simulink model "kundur_pv"  (R2023b)
settings: Solver=ode23tb  StartTime=0.0  StopTime=200  MaxStep=1/60  RelTol=1e-3
InitFcn:
  | SolarInverter_Params();
values from neighbouring files (symbols this model uses):
  Fnom = 60    [SolarInverter_Params.m]
  Pnom = 900e6    (= 900000000)    [SolarInverter_Params.m]
  reec_dbd1 = -0.1    [SolarInverter_Params.m]
  reec_dbd2 = 0.1    [SolarInverter_Params.m]
  reec_dPmax = 0.1    [SolarInverter_Params.m]
  reec_dPmin = -0.1    [SolarInverter_Params.m]
  reec_Imax = 1    [SolarInverter_Params.m]
  reec_Iqhl = 1.0    (= 1)    [SolarInverter_Params.m]
  reec_Iqll = -0.4    [SolarInverter_Params.m]
  reec_Kqi = 0.0    (= 0)    [SolarInverter_Params.m]
  reec_Kqp = 0    [SolarInverter_Params.m]
  reec_Kvi = 0.0    (= 0)    [SolarInverter_Params.m]
  reec_Kvp = 0.1    [SolarInverter_Params.m]
  reec_Pmax = 1.0    (= 1)    [SolarInverter_Params.m]
  reec_Pmin = 0    [SolarInverter_Params.m]
  reec_Qmax = 0.435    [SolarInverter_Params.m]
  reec_Qmin = -0.435    [SolarInverter_Params.m]
  reec_Tiq = 0.02    [SolarInverter_Params.m]
  reec_Tp = 0.02    [SolarInverter_Params.m]
  reec_Tpord = 0.1    [SolarInverter_Params.m]
  reec_Trv = 0.01    [SolarInverter_Params.m]
  reec_Vdip = 0.9    [SolarInverter_Params.m]
  reec_Vmax = 1.10    (= 1.1)    [SolarInverter_Params.m]
  reec_Vmin = 0.9    [SolarInverter_Params.m]
  reec_Vup = 1.15    [SolarInverter_Params.m]
  regc_Brkpt = 0.9    [SolarInverter_Params.m]
  regc_Iolim = -1.2    [SolarInverter_Params.m]
  regc_Iqrmax = 999.9    [SolarInverter_Params.m]
  regc_Iqrmin = -999.9    [SolarInverter_Params.m]
  regc_Ivpnt0 = 0.4    [SolarInverter_Params.m]
  regc_Ivpnt1 = 0.8    [SolarInverter_Params.m]
  regc_Khv = 0.0    (= 0)    [SolarInverter_Params.m]
  regc_Lvpl1 = 1.0    (= 1)    [SolarInverter_Params.m]
  regc_Lvplsw = 0    [SolarInverter_Params.m]
  regc_rrpwr = 10    [SolarInverter_Params.m]
  regc_Tfltr = 0.02    [SolarInverter_Params.m]
  regc_Tg = 0.1    [SolarInverter_Params.m]
  regc_Volim = 1.1    [SolarInverter_Params.m]
  regc_Zerox = 0.5    [SolarInverter_Params.m]
  repc_db1 = 0    [SolarInverter_Params.m]
  repc_Ddn = 20    [SolarInverter_Params.m]
  repc_Dup = 0    [SolarInverter_Params.m]
  repc_emax = 999    [SolarInverter_Params.m]
  repc_emin = -999    [SolarInverter_Params.m]
  repc_fdbd1 = 0.01*0    (= 0)    [SolarInverter_Params.m]
  repc_fdbd2 = -0.01*0    (= 0)    [SolarInverter_Params.m]
  repc_femax = 999    [SolarInverter_Params.m]
  repc_femin = -999    [SolarInverter_Params.m]
  repc_Kc = 0.05    [SolarInverter_Params.m]
  repc_Ki = 1.8    [SolarInverter_Params.m]
  repc_Kig = 0.5    [SolarInverter_Params.m]
  repc_Kp = 0.6    [SolarInverter_Params.m]
  repc_Kpg = 0.1    [SolarInverter_Params.m]
  repc_Pmax = 1    [SolarInverter_Params.m]
  repc_Pmin = 0    [SolarInverter_Params.m]
  repc_Qmax = 0.435    [SolarInverter_Params.m]
  repc_Qmin = -0.435    [SolarInverter_Params.m]
  repc_Rc = 0    [SolarInverter_Params.m]
  repc_Tfltr = 0.02    [SolarInverter_Params.m]
  repc_Tft = 0.5    [SolarInverter_Params.m]
  repc_Tfv = 0.8    [SolarInverter_Params.m]
  repc_Tlag = 0.2    [SolarInverter_Params.m]
  repc_Tp = 0.25    [SolarInverter_Params.m]
  repc_Vfrz = 0.7    [SolarInverter_Params.m]
  repc_Xc = 0    [SolarInverter_Params.m]
  Vnom = 230e3    (= 230000)    [SolarInverter_Params.m]
undefined symbols (not defined in the file or in its folder): D1, Delta, FrqControl, gcbh, j, k_fault, k_pulse, pfaref0, PFControl, PlantControl, PQPriority, Pref_pl, QControl, Qref_pl, QVControl, sps_rtmsupport, Vref_pl
libraries: powerlib_extras x24, simulink x13, spsLoadFlowBusLib x12, spsThreePhaseVIMeasurementLib x11, spsThreePhasePISectionLineLib x8, spsThreePhaseTransformerTwoWindingsLib x5, spsThreePhaseParallelRLCLoadLib x4, spsSynchronousMachinepuStandardLib x4, spsExcitationSystemLib x4, spsSteamTurbineandGovernorLib x4, spsGenericPowerSystemStabilizerLib x4, spsControlledCurrentSourceLib x2
(part 3 of 3)

== system kundur_pv/Renewable Grid-Connection/Break P Loop ==
  u : Inport
  Gain2 : Gain  Gain=1/tau
  Integrator2 : Integrator  InitialCondition=1
  Sum3 : Sum  Inputs=|+-
  to PU1 : Gain  Gain=toPU
  to PU7 : Gain  Gain=1/toPU
  y : Outport  VectorParamsAs1DForOutWhenUnconnected=off
  wires:
  Gain2/1 -> Integrator2/1
  Integrator2/1 -> to PU1/1, Sum3/2
  Sum3/1 -> Gain2/1
  u/1 -> to PU7/1
  to PU7/1 -> Sum3/1
  to PU1/1 -> y/1

== system kundur_pv/Renewable Grid-Connection/Break Q Loop ==
  u : Inport
  Gain2 : Gain  Gain=1/tau
  Integrator2 : Integrator
  Sum3 : Sum  Inputs=|+-
  to PU1 : Gain  Gain=toPU
  to PU7 : Gain  Gain=1/toPU
  y : Outport  VectorParamsAs1DForOutWhenUnconnected=off
  wires:
  to PU1/1 -> y/1
  to PU7/1 -> Sum3/1
  u/1 -> to PU7/1
  Sum3/1 -> Gain2/1
  Integrator2/1 -> Sum3/2, to PU1/1
  Gain2/1 -> Integrator2/1

== system kundur_pv/Renewable Grid-Connection/Break V Loop ==
  u : Inport
  Gain2 : Gain  Gain=1/tau
  Integrator2 : Integrator  InitialCondition=1
  Sum3 : Sum  Inputs=|+-
  to PU1 : Gain  Gain=toPU
  to PU7 : Gain  Gain=1/toPU
  y : Outport  VectorParamsAs1DForOutWhenUnconnected=off
  wires:
  Gain2/1 -> Integrator2/1
  Integrator2/1 -> to PU1/1, Sum3/2
  Sum3/1 -> Gain2/1
  u/1 -> to PU7/1
  to PU7/1 -> Sum3/1
  to PU1/1 -> y/1

== system kundur_pv/Renewable Grid-Connection/Clamping Integrator ==
  LVMax : Inport
  e : Inport  Port=2
  Constant : Constant  Value=-inf
  Constant1 : Constant  Value=0
  Integrator1 : Integrator  InitialCondition=1
  Saturation Dynamic : simulink/Discontinuities/Saturation Dynamic  OutMin=[]  OutMax=[]  OutDataTypeStr=Inherit: Same as second input  OutDataType=fixdt(1, 16)  OutScaling=2^-10  DoSatur=off
  Subsystem : Subsystem
  Switch1 : Switch  Criteria=u2 > Threshold  SaturateOnIntegerOverflow=off  InputSameDT=off
  u : Outport  VectorParamsAs1DForOutWhenUnconnected=off
  wires:
  Saturation Dynamic/1 -> u/1  "u"
  Subsystem/1(Clamp) -> Switch1/2
  Constant/1 -> Saturation Dynamic/3
  Switch1/1 -> Integrator1/1
  LVMax/1 -> Subsystem/3(ymax), Saturation Dynamic/1
  Integrator1/1 -> Subsystem/2(preSat), Saturation Dynamic/2
  e/1 -> Subsystem/1(preIntegrator), Switch1/3
  Constant1/1 -> Switch1/1

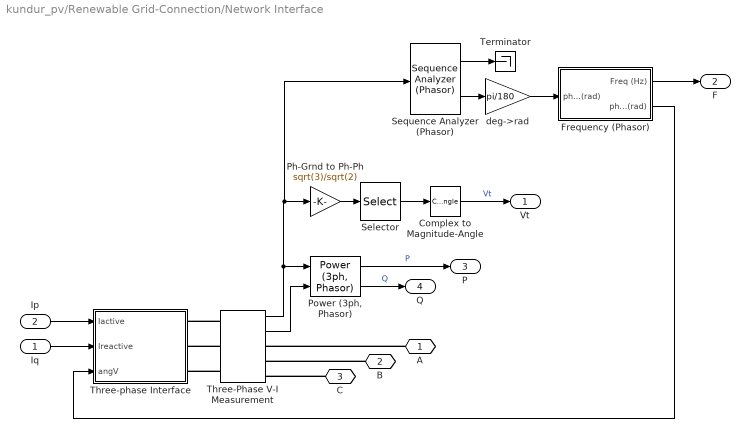
== system kundur_pv/Renewable Grid-Connection/Network Interface ==
  Iq : Inport
  Ip : Inport  Port=2
  Complex to Magnitude-Angle : ComplexToMagnitudeAngle  Output=Magnitude
  Frequency (Phasor) : Subsystem  DialogController=POWERSYS.PowerSysDialog  LoadFcn=sps_rtmsupport('LoadFcn', gcbh);  StartFcn=sps_rtmsupport('StartFcn', gcbh);  StopFcn=sps_rtmsupport('StopFcn', gcbh);  mask(Frequency (Phasor)){Fn=Fnom, T=0.01}
      mask prompts: Fn "Nominal frequency (Hz):"; T "Time constant T for derivative (s):"
      mask help:
      | Frequency is computed by derivative of input phase angle variation with respect to a synchronous phasor rotating at nominal frequency, using the following transfer function:
      |
      |      Hd = s / (1+T.s)
      |
      | The unwraped phase angle (without 2*pi discontinuities) is available at output 2.
      settings: CopyFcn=sps_rtmsupport('CopyFcn', gcbh);  DeleteFcn=sps_rtmsupport('DeleteFcn', gcbh);  UndoDeleteFcn=sps_rtmsupport('UndoDeleteFcn', gcbh);  ModelCloseFcn=sps_rtmsupport('ModelCloseFcn', gcbh);  PreSaveFcn=sps_rtmsupport('PreSaveFcn', gcbh);  PostSaveFcn=sps_rtmsupport('PostSaveFcn', gcbh);  NameChangeFcn=sps_rtmsupport('NameChangeFcn', gcbh);  PreCopyFcn=sps_rtmsupport('PreCopyFcn', gcbh);  OpenFcn=sps_rtmsupport('OpenFcn', gcbh, []);  CloseFcn=sps_rtmsupport('CloseFcn', gcbh);  PreDeleteFcn=sps_rtmsupport('PreDeleteFcn', gcbh);
      mask Help: helpview(psbhelp);
      mask Display:
      | port_label('input',1,'Phase (rad)')
      | port_label('output',1,'Freq (Hz)')
      | port_label('output',2,'\DeltaPhi (rad)', 'texmode', 'on')
  Ph-Grnd to Ph-Ph : Gain  Gain=sqrt(3)/sqrt(2)
  "Power (3ph, Phasor)" : spsPower3phPhasorLib/Power (3ph, Phasor)
      settings: LibrarySourceBlock=|
      | sps_lib/Sensors and Measurements/Power
      | (3ph, Phasor)
  Selector : Selector  InputPortWidth=3  IndexOptions=Index vector (dialog)  Indices=[1]  OutputSizes=1
  Sequence Analyzer (Phasor) : spsSequenceAnalyzerPhasorLib/Sequence Analyzer (Phasor)  seq=Positive
      settings: LibrarySourceBlock=|
      | sps_lib/Sensors and Measurements/Sequence Analyzer
      | (Phasor)
  Terminator : Terminator
  Three-Phase V-I Measurement : spsThreePhaseVIMeasurementLib/Three-Phase V-I Measurement  VoltageMeasurement=phase-to-ground  SetLabelV=off  LabelV=Vabc  Vpu=off  VpuLL=on  CurrentMeasurement=yes  SetLabelI=off  LabelI=Iabc  Ipu=off  Pbase=Pnom  Vbase=Vnom  OutputType=Complex  PhasorSimulation=on  PSBequivalent=0
  Three-phase Interface : Subsystem
  deg->rad : Gain  Gain=pi/180
  A : PMIOPort  Side=Right
  B : PMIOPort  Port=2  Side=Right
  C : PMIOPort  Port=3  Side=Right
  Vt : Outport  VectorParamsAs1DForOutWhenUnconnected=off
  F : Outport  Port=2  VectorParamsAs1DForOutWhenUnconnected=off
  P : Outport  Port=3  VectorParamsAs1DForOutWhenUnconnected=off
  Q : Outport  Port=4  VectorParamsAs1DForOutWhenUnconnected=off
  wires:
  Three-Phase V-I Measurement/1 -> "Power (3ph, Phasor)"/1, Sequence Analyzer (Phasor)/1, Ph-Grnd to Ph-Ph/1
  Three-Phase V-I Measurement/2 -> "Power (3ph, Phasor)"/2
  Selector/1 -> Complex to Magnitude-Angle/1
  Iq/1 -> Three-phase Interface/2(Ireactive)
  Ph-Grnd to Ph-Ph/1 -> Selector/1
  Complex to Magnitude-Angle/1 -> Vt/1  "Vt"
  "Power (3ph, Phasor)"/1 -> P/1  "P"
  Ip/1 -> Three-phase Interface/1(Iactive)
  "Power (3ph, Phasor)"/2 -> Q/1  "Q"
  Sequence Analyzer (Phasor)/2 -> deg->rad/1
  Sequence Analyzer (Phasor)/1 -> Terminator/1
  deg->rad/1 -> Frequency (Phasor)/1(phase (rad))
  Frequency (Phasor)/1(Freq (Hz)) -> F/1
  Frequency (Phasor)/2("phase (rad) ") -> Three-phase Interface/3(angV)
  connections:
  Three-Phase V-I Measurement/LConn3 -- Three-phase Interface/RConn3
  B/RConn1 -- Three-Phase V-I Measurement/RConn2
  Three-Phase V-I Measurement/LConn1 -- Three-phase Interface/RConn1
  A/RConn1 -- Three-Phase V-I Measurement/RConn1
  C/RConn1 -- Three-Phase V-I Measurement/RConn3
  Three-Phase V-I Measurement/LConn2 -- Three-phase Interface/RConn2

== system kundur_pv/Renewable Grid-Connection/Q Current Filter ==
  u : Inport
  1/(taus+1) : Subsystem  mask{tau=tau, vmax=vmax, vmin=vmin}
      mask prompts: tau "Time Constant"
  k : Gain  Gain=k
  y : Outport  VectorParamsAs1DForOutWhenUnconnected=off
  wires:
  1/(taus+1)/1(y) -> y/1
  u/1 -> k/1
  k/1 -> 1/(taus+1)/1(u)

== system kundur_pv/Renewable Grid-Connection/Voltage Filter ==
  u : Inport
  1/(taus+1) : Subsystem  mask{tau=tau, vmax=vmax, vmin=vmin}
      mask prompts: tau "Time Constant"
  k : Gain  Gain=k
  y : Outport  VectorParamsAs1DForOutWhenUnconnected=off
  wires:
  k/1 -> 1/(taus+1)/1(u)
  u/1 -> k/1
  1/(taus+1)/1(y) -> y/1

== system kundur_pv/Utility-scale Solar Electrical Controller/Active Power Filter ==
  u : Inport
  1/(taus+1) : Subsystem  mask{tau=tau, vmax=vmax, vmin=vmin}
      mask prompts: tau "Time Constant"
  k : Gain  Gain=k
  y : Outport  VectorParamsAs1DForOutWhenUnconnected=off
  wires:
  k/1 -> 1/(taus+1)/1(u)
  u/1 -> k/1
  1/(taus+1)/1(y) -> y/1

== system kundur_pv/Utility-scale Solar Electrical Controller/Current Controller ==
  e : Inport
  umax : Inport  Port=2
  umin : Inport  Port=3
  Vdip : Inport  Port=4
  Constant1 : Constant  Value=0
  Display : Display
  Gain : Gain  Gain=Kvp
  Gain1 : Gain  Gain=Kvi
  Integrator1 : Integrator
  OR : Logic  Operator=OR  AllPortsSameDT=off  OutDataTypeStr=boolean
  Saturation Dynamic : simulink/Discontinuities/Saturation Dynamic  OutMin=[]  OutMax=[]  OutDataTypeStr=Inherit: Same as second input  OutDataType=fixdt(1, 16)  OutScaling=2^-10  DoSatur=off
  Subsystem : Subsystem
  Sum1 : Sum  Inputs=++|
  Switch1 : Switch  Criteria=u2 > Threshold  SaturateOnIntegerOverflow=off  InputSameDT=off
  u : Outport  VectorParamsAs1DForOutWhenUnconnected=off
  wires:
  Gain/1 -> Sum1/1
  e/1 -> Gain/1, Gain1/1  "e"
  Constant1/1 -> Switch1/1
  umax/1 -> Subsystem/3(ymax), Saturation Dynamic/1
  Integrator1/1 -> Display/1, Sum1/2
  Gain1/1 -> Subsystem/1(preIntegrator), Switch1/3
  Switch1/1 -> Integrator1/1
  Saturation Dynamic/1 -> u/1  "u"
  Sum1/1 -> Subsystem/2(preSat), Saturation Dynamic/2
  umin/1 -> Subsystem/4(ymin), Saturation Dynamic/3
  Vdip/1 -> OR/1
  Subsystem/1(Clamp) -> OR/2
  OR/1 -> Switch1/2

== system kundur_pv/Utility-scale Solar Electrical Controller/Current Filter ==
  u : Inport
  Vflag : Inport  Port=2
  1/(taus+1) : Subsystem  mask{tau=tau, vmax=vmax, vmin=vmin}
      mask prompts: tau "Time Constant"
  k : Gain  Gain=k
  y : Outport  VectorParamsAs1DForOutWhenUnconnected=off
  wires:
  1/(taus+1)/1(y) -> y/1
  u/1 -> k/1
  k/1 -> 1/(taus+1)/1(u)
  Vflag/1 -> 1/(taus+1)/2(Vflag)

== system kundur_pv/Utility-scale Solar Electrical Controller/P Priority ==
  Ipcmd : Inport
  Constant8 : Constant  Value=Imax
  Sqrt : Sqrt
  Square : Math  Operator=square  SignedPower=on
  Square1 : Math  Operator=square  SignedPower=on
  Sum2 : Sum  Inputs=|+-
  Iqmax : Outport  VectorParamsAs1DForOutWhenUnconnected=off
  wires:
  Sqrt/1 -> Iqmax/1
  Sum2/1 -> Sqrt/1
  Constant8/1 -> Square/1
  Square1/1 -> Sum2/2
  Square/1 -> Sum2/1
  Ipcmd/1 -> Square1/1

== system kundur_pv/Utility-scale Solar Electrical Controller/Q Priority ==
  Iqcmd : Inport
  Constant8 : Constant  Value=Imax
  Sqrt : Sqrt
  Square : Math  Operator=square  SignedPower=on
  Square1 : Math  Operator=square  SignedPower=on
  Sum2 : Sum  Inputs=|+-
  Ipmax : Outport  VectorParamsAs1DForOutWhenUnconnected=off
  wires:
  Sqrt/1 -> Ipmax/1
  Sum2/1 -> Sqrt/1
  Constant8/1 -> Square/1
  Square1/1 -> Sum2/2
  Square/1 -> Sum2/1
  Iqcmd/1 -> Square1/1

== system kundur_pv/Utility-scale Solar Electrical Controller/Reference Power Filter ==
  u : Inport
  Vflag : Inport  Port=2
  1/(taus+1) : Subsystem  mask{tau=tau, vmax=vmax, vmin=vmin}
      mask prompts: tau "Time Constant"
  k : Gain  Gain=k
  y : Outport  VectorParamsAs1DForOutWhenUnconnected=off
  wires:
  Vflag/1 -> 1/(taus+1)/2(Vflag)
  k/1 -> 1/(taus+1)/1(u)
  u/1 -> k/1
  1/(taus+1)/1(y) -> y/1

== system kundur_pv/Utility-scale Solar Electrical Controller/Vref0 ==
  Constant6 : Constant  Value=0
  Init_Val : Integrator  InitialCondition=1
  Vref0 : Outport  VectorParamsAs1DForOutWhenUnconnected=off
  wires:
  Constant6/1 -> Init_Val/1
  Init_Val/1 -> Vref0/1

== system kundur_pv/Utility-scale Solar Electrical Controller/Vt Filter ==
  u : Inport
  1/(taus+1) : Subsystem  mask{tau=tau, vmax=vmax, vmin=vmin}
      mask prompts: tau "Time Constant"
  k : Gain  Gain=k
  y : Outport  VectorParamsAs1DForOutWhenUnconnected=off
  wires:
  k/1 -> 1/(taus+1)/1(u)
  u/1 -> k/1
  1/(taus+1)/1(y) -> y/1

== system kundur_pv/Utility-scale Solar Electrical Controller/pfaref ==
  Constant1 : Constant  Value=cos(pfaref0)
  Constant6 : Constant  Value=0
  Init_Val : Integrator
  Trigonometric Function : Trigonometry  Operator=acos
  pfaref : Outport  VectorParamsAs1DForOutWhenUnconnected=off
  wires:
  Constant6/1 -> Init_Val/1
  Constant1/1 -> Trigonometric Function/1
  Trigonometric Function/1 -> pfaref/1

== system kundur_pv/Utility-scale Solar Plant Controller/Lag Filter ==
  u : Inport
  1/(taus+1) : Subsystem  mask{tau=tau, vmax=vmax, vmin=vmin}
      mask prompts: tau "Time Constant"
  k : Gain  Gain=k
  y : Outport  VectorParamsAs1DForOutWhenUnconnected=off
  wires:
  k/1 -> 1/(taus+1)/1(u)
  u/1 -> k/1
  1/(taus+1)/1(y) -> y/1

== system kundur_pv/Utility-scale Solar Plant Controller/Lead-Lag ==
  note: disable integrator and pass through signal if tb is zero
  u : Inport
  Constant : Constant  Value=tb
  Gain : Gain  Gain=1/(tb+eps)
  Gain1 : Gain  Gain=ta
  Integrator : Integrator
  Sum : Sum  Inputs=|+-
  Sum1 : Sum  Inputs=++|
  Switch : Switch  Criteria=u2 > Threshold  SaturateOnIntegerOverflow=off  InputSameDT=off
  Switch1 : Switch  Criteria=u2 > Threshold  SaturateOnIntegerOverflow=off  InputSameDT=off
  y : Outport  VectorParamsAs1DForOutWhenUnconnected=off
  wires:
  Sum/1 -> Gain/1
  Gain/1 -> Switch/1, Gain1/1
  Gain1/1 -> Sum1/1
  Integrator/1 -> Sum1/2, Sum/2
  u/1 -> Switch1/3, Sum/1
  Constant/1 -> Switch1/2, Switch/3, Switch/2
  Switch/1 -> Integrator/1
  Sum1/1 -> Switch1/1
  Switch1/1 -> y/1

== system kundur_pv/Utility-scale Solar Plant Controller/P Filter ==
  u : Inport
  1/(taus+1) : Subsystem  mask{tau=tau, vmax=vmax, vmin=vmin}
      mask prompts: tau "Time Constant"
  k : Gain  Gain=k
  y : Outport  VectorParamsAs1DForOutWhenUnconnected=off
  wires:
  k/1 -> 1/(taus+1)/1(u)
  u/1 -> k/1
  1/(taus+1)/1(y) -> y/1

== system kundur_pv/Utility-scale Solar Plant Controller/Q Filter ==
  u : Inport
  1/(taus+1) : Subsystem  mask{tau=tau, vmax=vmax, vmin=vmin}
      mask prompts: tau "Time Constant"
  k : Gain  Gain=k
  y : Outport  VectorParamsAs1DForOutWhenUnconnected=off
  wires:
  k/1 -> 1/(taus+1)/1(u)
  u/1 -> k/1
  1/(taus+1)/1(y) -> y/1

== system kundur_pv/Utility-scale Solar Plant Controller/Reactive Power Controller ==
  e : Inport
  Frz : Inport  Port=2
  Constant : Constant  Value=Qmax
  Constant1 : Constant  Value=0
  Constant2 : Constant  Value=Qmin
  Display2 : Display
  Gain : Gain  Gain=Kp
  Gain1 : Gain  Gain=Ki
  Integrator1 : Integrator
  OR : Logic  Operator=OR  AllPortsSameDT=off  OutDataTypeStr=boolean
  Saturation Dynamic : simulink/Discontinuities/Saturation Dynamic  OutMin=[]  OutMax=[]  OutDataTypeStr=Inherit: Same as second input  OutDataType=fixdt(1, 16)  OutScaling=2^-10  DoSatur=off
  Subsystem : Subsystem
  Sum1 : Sum  Inputs=++|
  Switch1 : Switch  Criteria=u2 > Threshold  SaturateOnIntegerOverflow=off  InputSameDT=off
  u : Outport  VectorParamsAs1DForOutWhenUnconnected=off
  wires:
  OR/1 -> Switch1/2
  Subsystem/1(Clamp) -> OR/2
  Frz/1 -> OR/1
  Constant2/1 -> Saturation Dynamic/3, Subsystem/4(ymin)
  Sum1/1 -> Display2/1, Saturation Dynamic/2, Subsystem/2(preSat)
  Saturation Dynamic/1 -> u/1  "u"
  Switch1/1 -> Integrator1/1
  Gain1/1 -> Switch1/3, Subsystem/1(preIntegrator)
  Integrator1/1 -> Sum1/2
  Constant/1 -> Saturation Dynamic/1, Subsystem/3(ymax)
  Constant1/1 -> Switch1/1
  e/1 -> Gain1/1, Gain/1  "e"
  Gain/1 -> Sum1/1

== system kundur_pv/Utility-scale Solar Plant Controller/Subsystem ==
  Ibranch : Inport
  Vreg : Inport  Port=2
  Complex to Magnitude : ComplexToMagnitudeAngle  Output=Magnitude
  Gain : Gain  Gain=Rc
  Gain1 : Gain  Gain=j*Xc
  Sum : Sum  Inputs=|++
  Sum1 : Sum  Inputs=|-+
  Ve : Outport  VectorParamsAs1DForOutWhenUnconnected=off
  wires:
  Ibranch/1 -> Gain/1, Gain1/1
  Gain/1 -> Sum/1
  Vreg/1 -> Sum1/2
  Sum/1 -> Sum1/1
  Gain1/1 -> Sum/2
  Sum1/1 -> Complex to Magnitude/1
  Complex to Magnitude/1 -> Ve/1  "Ve"

== system kundur_pv/Utility-scale Solar Plant Controller/Vcomp Filter ==
  u : Inport
  1/(taus+1) : Subsystem  mask{tau=tau, vmax=vmax, vmin=vmin}
      mask prompts: tau "Time Constant"
  k : Gain  Gain=k
  y : Outport  VectorParamsAs1DForOutWhenUnconnected=off
  wires:
  k/1 -> 1/(taus+1)/1(u)
  u/1 -> k/1
  1/(taus+1)/1(y) -> y/1

== system kundur_pv/Renewable Grid-Connection/Clamping Integrator/Subsystem ==
  preIntegrator : Inport
  preSat : Inport  Port=2
  ymax : Inport  Port=3
  AND1 : Logic  AllPortsSameDT=off  OutDataTypeStr=boolean
  Constant : Constant  Value=-inf
  Data Type Conversion : DataTypeConversion  OutDataTypeStr=int8  SaturateOnIntegerOverflow=off  RndMeth=Floor
  Data Type Conversion1 : DataTypeConversion  OutDataTypeStr=int8  SaturateOnIntegerOverflow=off  RndMeth=Floor
  Dead Zone Dynamic : simulink/Discontinuities/Dead Zone Dynamic
  Equal1 : RelationalOperator  Operator===  OutDataTypeStr=boolean  RndMeth=Simplest  InputSameDT=off
  Gain2 : Gain  Gain=0
  Memory1 : Memory
  Relational Operator : RelationalOperator  Operator=~=  OutDataTypeStr=boolean  RndMeth=Simplest  InputSameDT=off
  Sign : Signum
  Sign1 : Signum
  Clamp : Outport  VectorParamsAs1DForOutWhenUnconnected=off
  wires:
  Sign/1 -> Data Type Conversion/1
  AND1/1 -> Memory1/1
  Dead Zone Dynamic/1 -> Relational Operator/2, Sign/1
  Data Type Conversion/1 -> Equal1/1
  Gain2/1 -> Relational Operator/1
  Equal1/1 -> AND1/2
  preSat/1 -> Dead Zone Dynamic/2, Gain2/1
  Relational Operator/1 -> AND1/1
  Sign1/1 -> Data Type Conversion1/1
  preIntegrator/1 -> Sign1/1
  Data Type Conversion1/1 -> Equal1/2
  ymax/1 -> Dead Zone Dynamic/1
  Constant/1 -> Dead Zone Dynamic/3
  Memory1/1 -> Clamp/1  "Clamp"

== system kundur_pv/Renewable Grid-Connection/Network Interface/Frequency (Phasor) ==
  phase (rad) : Inport
  " Wn" : Constant  Value=Fn*2*pi
  Add : Sum
  IC : InitialCondition  Commented=through  Value=0
  Unit Delay : UnitDelay  SampleTime=-1  HasFrameUpgradeWarning=on
  Unit Delay1 : UnitDelay  SampleTime=-1  HasFrameUpgradeWarning=on
  derivative : TransferFcn  Numerator="[1  0]"  Denominator="[T  1]"
  if structure : MATLAB Function  TreatAsAtomicUnit=on
  rad/s to Hz : Gain  Gain=1/(2*pi)
  Freq (Hz) : Outport  VectorParamsAs1DForOutWhenUnconnected=off
  "phase (rad) " : Outport  Port=2  VectorParamsAs1DForOutWhenUnconnected=off
  wires:
  Add/1 -> rad/s to Hz/1
  if structure/1(y) -> Unit Delay/1, derivative/1, "phase (rad) "/1
  rad/s to Hz/1 -> Freq (Hz)/1
  derivative/1 -> Add/1
  " Wn"/1 -> Add/2
  IC/1 -> if structure/1(phase)
  Unit Delay/1 -> if structure/3(y_old)
  Unit Delay1/1 -> if structure/2(phase_old)
  phase (rad)/1 -> Unit Delay1/1, IC/1

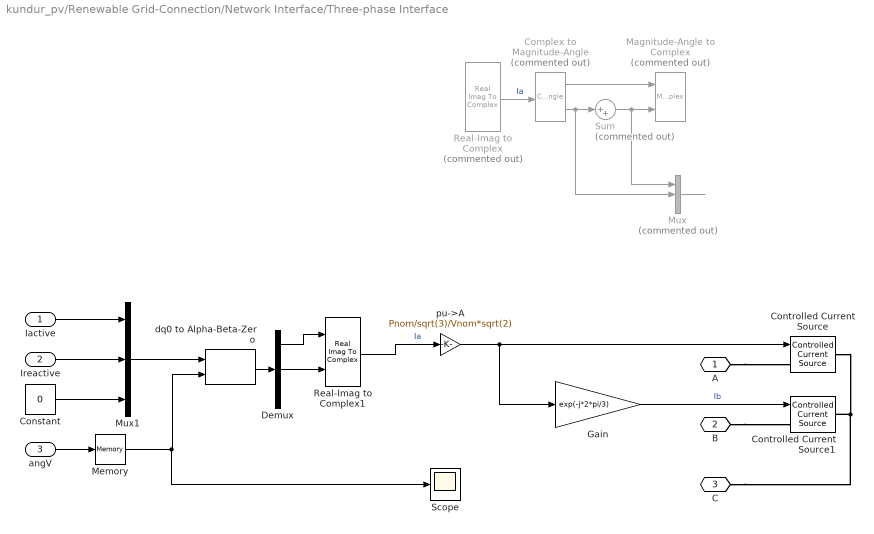
== system kundur_pv/Renewable Grid-Connection/Network Interface/Three-phase Interface ==
  Iactive : Inport
  Ireactive : Inport  Port=2
  angV : Inport  Port=3
  Complex to Magnitude-Angle : ComplexToMagnitudeAngle  Commented=on
  Constant : Constant  Value=0
  Controlled Current Source : spsControlledCurrentSourceLib/Controlled Current Source  Initialize=on  Source_Type=AC  Amplitude=-1*Pnom/sqrt(3)/Vnom*sqrt(2)  Phase=0  Frequency=Fnom  Measurements=None
  Controlled Current Source1 : spsControlledCurrentSourceLib/Controlled Current Source  Initialize=on  Source_Type=AC  Amplitude=-1*Pnom/sqrt(3)/Vnom*sqrt(2)  Phase=120  Frequency=Fnom  Measurements=None
  Demux : Demux  Outputs=3
  Gain : Gain  Gain=exp(-j*2*pi/3)
  Magnitude-Angle to Complex : MagnitudeAngleToComplex  Commented=on
  Memory : Memory  InitialCondition=0.1
  Mux : Mux  Commented=on  Inputs=3
  Mux1 : Mux  Inputs=3
  Real-Imag to Complex : RealImagToComplex  Commented=on
  Real-Imag to Complex1 : RealImagToComplex
  Scope : Scope
  Sum : Sum  Commented=on  Inputs=|++
  dq0 to Alpha-Beta-Zero : spsdq0toAlphaBetaZeroLib/dq0 to Alpha-Beta-Zero  Alignment=Aligned with phase A axis
  "pu->A " : Gain  Gain=Pnom/sqrt(3)/Vnom*sqrt(2)  SaturateOnIntegerOverflow=on  OutDataTypeStr=Inherit: Same as input  ParamDataTypeStr=Inherit: Same as input
  A : PMIOPort  Side=Right
  B : PMIOPort  Port=2  Side=Right
  C : PMIOPort  Port=3  Side=Right
  wires:
  Gain/1 -> Controlled Current Source1/1  "Ib"
  Real-Imag to Complex/1 -> Complex to Magnitude-Angle/1  "Ia"
  Complex to Magnitude-Angle/1 -> Magnitude-Angle to Complex/1
  Complex to Magnitude-Angle/2 -> Mux/2, Sum/1
  Sum/1 -> Mux/1, Magnitude-Angle to Complex/2
  "pu->A "/1 -> Gain/1, Controlled Current Source/1
  Mux/1 -> ?
  angV/1 -> Memory/1
  Iactive/1 -> Mux1/1
  Ireactive/1 -> Mux1/2
  Constant/1 -> Mux1/3
  Mux1/1 -> dq0 to Alpha-Beta-Zero/1
  dq0 to Alpha-Beta-Zero/1 -> Demux/1
  Demux/2 -> Real-Imag to Complex1/2
  Demux/1 -> Real-Imag to Complex1/1
  Real-Imag to Complex1/1 -> "pu->A "/1  "Ia"
  Memory/1 -> Scope/1, dq0 to Alpha-Beta-Zero/2
  connections:
  Controlled Current Source/RConn1 -- C/RConn1 -- Controlled Current Source1/RConn1
  A/RConn1 -- Controlled Current Source/LConn1
  B/RConn1 -- Controlled Current Source1/LConn1

== system kundur_pv/Renewable Grid-Connection/Q Current Filter/1//(taus+1) ==
  note: disable integrator and pass through signal if tau is zero
  u : Inport
  Constant : Constant  Value=tau
  Gain1 : Gain  Gain=1/(tau+eps)  SaturateOnIntegerOverflow=on  OutDataTypeStr=Inherit: Same as input  ParamDataTypeStr=Inherit: Same as input
  Integrator : Integrator  LimitOutput=on  UpperSaturationLimit=vmax  LowerSaturationLimit=vmin
  Sum : Sum  Inputs=|+-  InputSameDT=on  SaturateOnIntegerOverflow=on  OutDataTypeStr=Inherit: Same as first input
  Switch : Switch  Criteria=u2 > Threshold  SaturateOnIntegerOverflow=off  InputSameDT=off
  Switch1 : Switch  Criteria=u2 > Threshold  SaturateOnIntegerOverflow=off  InputSameDT=off
  y : Outport  VectorParamsAs1DForOutWhenUnconnected=off
  wires:
  Switch1/1 -> y/1
  Switch/1 -> Integrator/1
  Gain1/1 -> Switch/1
  Constant/1 -> Switch/2, Switch1/2, Switch/3
  Integrator/1 -> Switch1/1, Sum/2
  Sum/1 -> Gain1/1
  u/1 -> Sum/1, Switch1/3

== system kundur_pv/Renewable Grid-Connection/Voltage Filter/1//(taus+1) ==
  note: disable integrator and pass through signal if tau is zero
  u : Inport
  Constant : Constant  Value=tau
  Gain1 : Gain  Gain=1/(tau+eps)  SaturateOnIntegerOverflow=on  OutDataTypeStr=Inherit: Same as input  ParamDataTypeStr=Inherit: Same as input
  Integrator : Integrator  InitialCondition=1  LimitOutput=on  UpperSaturationLimit=vmax  LowerSaturationLimit=vmin
  Sum : Sum  Inputs=|+-  InputSameDT=on  SaturateOnIntegerOverflow=on  OutDataTypeStr=Inherit: Same as first input
  Switch : Switch  Criteria=u2 > Threshold  SaturateOnIntegerOverflow=off  InputSameDT=off
  Switch1 : Switch  Criteria=u2 > Threshold  SaturateOnIntegerOverflow=off  InputSameDT=off
  y : Outport  VectorParamsAs1DForOutWhenUnconnected=off
  wires:
  Sum/1 -> Gain1/1
  Integrator/1 -> Sum/2, Switch1/1
  Constant/1 -> Switch/3, Switch1/2, Switch/2
  Gain1/1 -> Switch/1
  Switch/1 -> Integrator/1
  Switch1/1 -> y/1
  u/1 -> Switch1/3, Sum/1

== system kundur_pv/Utility-scale Solar Electrical Controller/Active Power Filter/1//(taus+1) ==
  note: disable integrator and pass through signal if tau is zero
  u : Inport
  Constant : Constant  Value=tau
  Gain1 : Gain  Gain=1/(tau+eps)  SaturateOnIntegerOverflow=on  OutDataTypeStr=Inherit: Same as input  ParamDataTypeStr=Inherit: Same as input
  Integrator : Integrator  InitialCondition=1  LimitOutput=on  UpperSaturationLimit=vmax  LowerSaturationLimit=vmin
  Sum : Sum  Inputs=|+-  InputSameDT=on  SaturateOnIntegerOverflow=on  OutDataTypeStr=Inherit: Same as first input
  Switch : Switch  Criteria=u2 > Threshold  SaturateOnIntegerOverflow=off  InputSameDT=off
  Switch1 : Switch  Criteria=u2 > Threshold  SaturateOnIntegerOverflow=off  InputSameDT=off
  y : Outport  VectorParamsAs1DForOutWhenUnconnected=off
  wires:
  u/1 -> Switch1/3, Sum/1
  Sum/1 -> Gain1/1
  Integrator/1 -> Sum/2, Switch1/1
  Constant/1 -> Switch/3, Switch1/2, Switch/2
  Gain1/1 -> Switch/1
  Switch/1 -> Integrator/1
  Switch1/1 -> y/1

== system kundur_pv/Utility-scale Solar Electrical Controller/Current Controller/Subsystem ==
  preIntegrator : Inport
  preSat : Inport  Port=2
  ymax : Inport  Port=3
  ymin : Inport  Port=4
  AND1 : Logic  AllPortsSameDT=off  OutDataTypeStr=boolean
  Data Type Conversion : DataTypeConversion  OutDataTypeStr=int8  SaturateOnIntegerOverflow=off  RndMeth=Floor
  Data Type Conversion1 : DataTypeConversion  OutDataTypeStr=int8  SaturateOnIntegerOverflow=off  RndMeth=Floor
  Dead Zone Dynamic : simulink/Discontinuities/Dead Zone Dynamic
  Equal1 : RelationalOperator  Operator===  OutDataTypeStr=boolean  RndMeth=Simplest  InputSameDT=off
  Gain2 : Gain  Gain=0
  Memory1 : Memory
  Relational Operator : RelationalOperator  Operator=~=  OutDataTypeStr=boolean  RndMeth=Simplest  InputSameDT=off
  Sign : Signum
  Sign1 : Signum
  Clamp : Outport  VectorParamsAs1DForOutWhenUnconnected=off
  wires:
  Sign/1 -> Data Type Conversion/1
  AND1/1 -> Memory1/1
  Dead Zone Dynamic/1 -> Relational Operator/2, Sign/1
  Data Type Conversion/1 -> Equal1/1
  Gain2/1 -> Relational Operator/1
  Equal1/1 -> AND1/2
  preSat/1 -> Dead Zone Dynamic/2, Gain2/1
  Relational Operator/1 -> AND1/1
  Sign1/1 -> Data Type Conversion1/1
  preIntegrator/1 -> Sign1/1
  Data Type Conversion1/1 -> Equal1/2
  ymax/1 -> Dead Zone Dynamic/1
  ymin/1 -> Dead Zone Dynamic/3
  Memory1/1 -> Clamp/1  "Clamp"

== system kundur_pv/Utility-scale Solar Electrical Controller/Current Filter/1//(taus+1) ==
  note: disable integrator and pass through signal if tau is zero
  u : Inport
  Vflag : Inport  Port=2
  Constant : Constant  Value=tau
  Constant1 : Constant  Value=0
  Gain1 : Gain  Gain=1/(tau+eps)  SaturateOnIntegerOverflow=on  OutDataTypeStr=Inherit: Same as input  ParamDataTypeStr=Inherit: Same as input
  Integrator : Integrator  LimitOutput=on  UpperSaturationLimit=vmax  LowerSaturationLimit=vmin
  Subsystem : Subsystem
  Sum : Sum  Inputs=|+-  InputSameDT=on  SaturateOnIntegerOverflow=on  OutDataTypeStr=Inherit: Same as first input
  Switch : Switch  Criteria=u2 > Threshold  SaturateOnIntegerOverflow=off  InputSameDT=off
  Switch1 : Switch  Criteria=u2 > Threshold  SaturateOnIntegerOverflow=off  InputSameDT=off
  y : Outport  VectorParamsAs1DForOutWhenUnconnected=off
  wires:
  Switch1/1 -> y/1
  Switch/1 -> Integrator/1
  Gain1/1 -> Switch/1
  Constant/1 -> Switch1/2, Subsystem/1(tau)
  Integrator/1 -> Switch1/1, Sum/2
  Sum/1 -> Gain1/1
  u/1 -> Sum/1, Switch1/3
  Constant1/1 -> Switch/3
  Subsystem/1(Out1) -> Switch/2
  Vflag/1 -> Subsystem/2(Vflag)

== system kundur_pv/Utility-scale Solar Electrical Controller/Reference Power Filter/1//(taus+1) ==
  note: disable integrator and pass through signal if tau is zero
  u : Inport
  Vflag : Inport  Port=2
  Constant : Constant  Value=tau
  Constant1 : Constant  Value=0
  Gain1 : Gain  Gain=1/(tau+eps)  SaturateOnIntegerOverflow=on  OutDataTypeStr=Inherit: Same as input  ParamDataTypeStr=Inherit: Same as input
  Integrator : Integrator  InitialCondition=0.999  LimitOutput=on  UpperSaturationLimit=vmax  LowerSaturationLimit=vmin
  Subsystem : Subsystem
  Sum : Sum  Inputs=|+-  InputSameDT=on  SaturateOnIntegerOverflow=on  OutDataTypeStr=Inherit: Same as first input
  Switch : Switch  Criteria=u2 > Threshold  SaturateOnIntegerOverflow=off  InputSameDT=off
  Switch1 : Switch  Criteria=u2 > Threshold  SaturateOnIntegerOverflow=off  InputSameDT=off
  y : Outport  VectorParamsAs1DForOutWhenUnconnected=off
  wires:
  Vflag/1 -> Subsystem/2(Vflag)
  Subsystem/1(Out1) -> Switch/2
  Constant1/1 -> Switch/3
  u/1 -> Switch1/3, Sum/1
  Sum/1 -> Gain1/1
  Integrator/1 -> Sum/2, Switch1/1
  Constant/1 -> Subsystem/1(tau), Switch1/2
  Gain1/1 -> Switch/1
  Switch/1 -> Integrator/1
  Switch1/1 -> y/1

== system kundur_pv/Utility-scale Solar Electrical Controller/Vt Filter/1//(taus+1) ==
  note: disable integrator and pass through signal if tau is zero
  u : Inport
  Constant : Constant  Value=tau
  Gain1 : Gain  Gain=1/(tau+eps)  SaturateOnIntegerOverflow=on  OutDataTypeStr=Inherit: Same as input  ParamDataTypeStr=Inherit: Same as input
  Integrator : Integrator  InitialCondition=1  LimitOutput=on  UpperSaturationLimit=vmax  LowerSaturationLimit=vmin
  Sum : Sum  Inputs=|+-  InputSameDT=on  SaturateOnIntegerOverflow=on  OutDataTypeStr=Inherit: Same as first input
  Switch : Switch  Criteria=u2 > Threshold  SaturateOnIntegerOverflow=off  InputSameDT=off
  Switch1 : Switch  Criteria=u2 > Threshold  SaturateOnIntegerOverflow=off  InputSameDT=off
  y : Outport  VectorParamsAs1DForOutWhenUnconnected=off
  wires:
  u/1 -> Switch1/3, Sum/1
  Sum/1 -> Gain1/1
  Integrator/1 -> Sum/2, Switch1/1
  Constant/1 -> Switch/3, Switch1/2, Switch/2
  Gain1/1 -> Switch/1
  Switch/1 -> Integrator/1
  Switch1/1 -> y/1

== system kundur_pv/Utility-scale Solar Plant Controller/Lag Filter/1//(taus+1) ==
  note: disable integrator and pass through signal if tau is zero
  u : Inport
  Constant : Constant  Value=tau
  Gain1 : Gain  Gain=1/(tau+eps)  SaturateOnIntegerOverflow=on  OutDataTypeStr=Inherit: Same as input  ParamDataTypeStr=Inherit: Same as input
  Integrator : Integrator  InitialCondition=1  LimitOutput=on  UpperSaturationLimit=vmax  LowerSaturationLimit=vmin
  Sum : Sum  Inputs=|+-  InputSameDT=on  SaturateOnIntegerOverflow=on  OutDataTypeStr=Inherit: Same as first input
  Switch : Switch  Criteria=u2 > Threshold  SaturateOnIntegerOverflow=off  InputSameDT=off
  Switch1 : Switch  Criteria=u2 > Threshold  SaturateOnIntegerOverflow=off  InputSameDT=off
  y : Outport  VectorParamsAs1DForOutWhenUnconnected=off
  wires:
  u/1 -> Switch1/3, Sum/1
  Sum/1 -> Gain1/1
  Integrator/1 -> Sum/2, Switch1/1
  Constant/1 -> Switch/3, Switch1/2, Switch/2
  Gain1/1 -> Switch/1
  Switch/1 -> Integrator/1
  Switch1/1 -> y/1

== system kundur_pv/Utility-scale Solar Plant Controller/P Filter/1//(taus+1) ==
  note: disable integrator and pass through signal if tau is zero
  u : Inport
  Constant : Constant  Value=tau
  Gain1 : Gain  Gain=1/(tau+eps)  SaturateOnIntegerOverflow=on  OutDataTypeStr=Inherit: Same as input  ParamDataTypeStr=Inherit: Same as input
  Integrator : Integrator  InitialCondition=1  LimitOutput=on  UpperSaturationLimit=vmax  LowerSaturationLimit=vmin
  Sum : Sum  Inputs=|+-  InputSameDT=on  SaturateOnIntegerOverflow=on  OutDataTypeStr=Inherit: Same as first input
  Switch : Switch  Criteria=u2 > Threshold  SaturateOnIntegerOverflow=off  InputSameDT=off
  Switch1 : Switch  Criteria=u2 > Threshold  SaturateOnIntegerOverflow=off  InputSameDT=off
  y : Outport  VectorParamsAs1DForOutWhenUnconnected=off
  wires:
  u/1 -> Switch1/3, Sum/1
  Sum/1 -> Gain1/1
  Integrator/1 -> Sum/2, Switch1/1
  Constant/1 -> Switch/3, Switch1/2, Switch/2
  Gain1/1 -> Switch/1
  Switch/1 -> Integrator/1
  Switch1/1 -> y/1

== system kundur_pv/Utility-scale Solar Plant Controller/Q Filter/1//(taus+1) ==
  note: disable integrator and pass through signal if tau is zero
  u : Inport
  Constant : Constant  Value=tau
  Gain1 : Gain  Gain=1/(tau+eps)  SaturateOnIntegerOverflow=on  OutDataTypeStr=Inherit: Same as input  ParamDataTypeStr=Inherit: Same as input
  Integrator : Integrator  LimitOutput=on  UpperSaturationLimit=vmax  LowerSaturationLimit=vmin
  Sum : Sum  Inputs=|+-  InputSameDT=on  SaturateOnIntegerOverflow=on  OutDataTypeStr=Inherit: Same as first input
  Switch : Switch  Criteria=u2 > Threshold  SaturateOnIntegerOverflow=off  InputSameDT=off
  Switch1 : Switch  Criteria=u2 > Threshold  SaturateOnIntegerOverflow=off  InputSameDT=off
  y : Outport  VectorParamsAs1DForOutWhenUnconnected=off
  wires:
  u/1 -> Switch1/3, Sum/1
  Sum/1 -> Gain1/1
  Integrator/1 -> Sum/2, Switch1/1
  Constant/1 -> Switch/3, Switch1/2, Switch/2
  Gain1/1 -> Switch/1
  Switch/1 -> Integrator/1
  Switch1/1 -> y/1

== system kundur_pv/Utility-scale Solar Plant Controller/Reactive Power Controller/Subsystem ==
  preIntegrator : Inport
  preSat : Inport  Port=2
  ymax : Inport  Port=3
  ymin : Inport  Port=4
  AND1 : Logic  AllPortsSameDT=off  OutDataTypeStr=boolean
  Data Type Conversion : DataTypeConversion  OutDataTypeStr=int8  SaturateOnIntegerOverflow=off  RndMeth=Floor
  Data Type Conversion1 : DataTypeConversion  OutDataTypeStr=int8  SaturateOnIntegerOverflow=off  RndMeth=Floor
  Dead Zone Dynamic : simulink/Discontinuities/Dead Zone Dynamic
  Equal1 : RelationalOperator  Operator===  OutDataTypeStr=boolean  RndMeth=Simplest  InputSameDT=off
  Gain2 : Gain  Gain=0
  Memory1 : Memory
  Relational Operator : RelationalOperator  Operator=~=  OutDataTypeStr=boolean  RndMeth=Simplest  InputSameDT=off
  Sign : Signum
  Sign1 : Signum
  Clamp : Outport  VectorParamsAs1DForOutWhenUnconnected=off
  wires:
  Memory1/1 -> Clamp/1  "Clamp"
  ymin/1 -> Dead Zone Dynamic/3
  ymax/1 -> Dead Zone Dynamic/1
  Data Type Conversion1/1 -> Equal1/2
  preIntegrator/1 -> Sign1/1
  Sign1/1 -> Data Type Conversion1/1
  Relational Operator/1 -> AND1/1
  preSat/1 -> Gain2/1, Dead Zone Dynamic/2
  Equal1/1 -> AND1/2
  Gain2/1 -> Relational Operator/1
  Data Type Conversion/1 -> Equal1/1
  Dead Zone Dynamic/1 -> Sign/1, Relational Operator/2
  AND1/1 -> Memory1/1
  Sign/1 -> Data Type Conversion/1

== system kundur_pv/Utility-scale Solar Plant Controller/Vcomp Filter/1//(taus+1) ==
  note: disable integrator and pass through signal if tau is zero
  u : Inport
  Constant : Constant  Value=tau
  Gain1 : Gain  Gain=1/(tau+eps)  SaturateOnIntegerOverflow=on  OutDataTypeStr=Inherit: Same as input  ParamDataTypeStr=Inherit: Same as input
  Integrator : Integrator  InitialCondition=1  LimitOutput=on  UpperSaturationLimit=vmax  LowerSaturationLimit=vmin
  Sum : Sum  Inputs=|+-  InputSameDT=on  SaturateOnIntegerOverflow=on  OutDataTypeStr=Inherit: Same as first input
  Switch : Switch  Criteria=u2 > Threshold  SaturateOnIntegerOverflow=off  InputSameDT=off
  Switch1 : Switch  Criteria=u2 > Threshold  SaturateOnIntegerOverflow=off  InputSameDT=off
  y : Outport  VectorParamsAs1DForOutWhenUnconnected=off
  wires:
  u/1 -> Switch1/3, Sum/1
  Sum/1 -> Gain1/1
  Integrator/1 -> Sum/2, Switch1/1
  Constant/1 -> Switch/3, Switch1/2, Switch/2
  Gain1/1 -> Switch/1
  Switch/1 -> Integrator/1
  Switch1/1 -> y/1

== system kundur_pv/Utility-scale Solar Electrical Controller/Current Filter/1//(taus+1)/Subsystem ==
  tau : Inport
  Vflag : Inport  Port=2
  AND : Logic  AllPortsSameDT=off  OutDataTypeStr=boolean
  Compare To Zero : simulink/Logic and Bit Operations/Compare To Zero  relop=>  OutDataTypeStr=boolean
  NOT : Logic  Operator=NOT  AllPortsSameDT=off  OutDataTypeStr=boolean
  Out1 : Outport  VectorParamsAs1DForOutWhenUnconnected=off
  wires:
  NOT/1 -> AND/2
  tau/1 -> Compare To Zero/1
  AND/1 -> Out1/1
  Compare To Zero/1 -> AND/1
  Vflag/1 -> NOT/1

== system kundur_pv/Utility-scale Solar Electrical Controller/Reference Power Filter/1//(taus+1)/Subsystem ==
  tau : Inport
  Vflag : Inport  Port=2
  AND : Logic  AllPortsSameDT=off  OutDataTypeStr=boolean
  Compare To Zero : simulink/Logic and Bit Operations/Compare To Zero  relop=>  OutDataTypeStr=boolean
  NOT : Logic  Operator=NOT  AllPortsSameDT=off  OutDataTypeStr=boolean
  Out1 : Outport  VectorParamsAs1DForOutWhenUnconnected=off
  wires:
  Vflag/1 -> NOT/1
  Compare To Zero/1 -> AND/1
  AND/1 -> Out1/1
  tau/1 -> Compare To Zero/1
  NOT/1 -> AND/2

== matlab function kundur_pv/Renewable Grid-Connection/Network Interface/Frequency (Phasor)/if structure ==
  data: phase input; phase_old input; y output; y_old input
function y = fcn(phase,phase_old,y_old)

u = phase-phase_old;
if u > 0.9*2*pi
    y=y_old+u-(2*pi);
elseif u < -(0.9*2*pi)
    y=y_old+u+(2*pi);
else
    y=y_old+u(1);
end

== stateflow chart kundur_pv/Local and Plant Level Controller ==
  state ReactivePower [parallel]
    Mode.VcompFlag = 1;
    settings: executionOrder=1
    state V_Control
      Mode.PfFlag = 0;
      state PlantLevel
        Mode.QFlag = 0;
        Mode.RefFlag = 1;
      state LocalLevel
        Mode.VFlag = 0;
        Mode.QFlag = 1;
      (default) -> ReactivePower.V_Control.PlantLevel
      ReactivePower.V_Control.LocalLevel -> ReactivePower.V_Control.PlantLevel : [PlantControl == 1]
      ReactivePower.V_Control.PlantLevel -> ReactivePower.V_Control.LocalLevel : [PlantControl == 0]
    state Q_Control
      Mode.PfFlag = 0;
      Mode.VFlag = 1;
      state PlantLevel
        Mode.QFlag = 0;
        Mode.RefFlag = 0;
      state LocalLevel
        Mode.QFlag = 0;
      (default) -> ReactivePower.Q_Control.PlantLevel
      ReactivePower.Q_Control.LocalLevel -> ReactivePower.Q_Control.PlantLevel : [PlantControl == 1]
      ReactivePower.Q_Control.PlantLevel -> ReactivePower.Q_Control.LocalLevel : [PlantControl == 0]
    state PowerFactor
      Mode.PfFlag = 1;
      Mode.QFlag = 0;
    (default) -> V_Control
    Q_Control -> V_Control [order 1] : [QControl == 0]
    V_Control -> Q_Control [order 1] : [QControl == 1]
    PowerFactor -> Q_Control [order 2] : [PFControl == 0 && ...
        | QControl == 1]
    Q_Control -> PowerFactor [order 2] : [PFControl == 1]
    PowerFactor -> V_Control [order 1] : [PFControl == 0 && ...
        | QControl == 0]
    V_Control -> PowerFactor [order 2] : [PFControl == 1]
  state ActivePower [parallel]
    settings: executionOrder=2
    state NoGovenorResponse
      Mode.FrqFlag = 0;
    state GovernorResponse
      Mode.FrqFlag = 1;
    (default) -> GovernorResponse
    GovernorResponse -> NoGovenorResponse : [FrqControl == 0]
    NoGovenorResponse -> GovernorResponse : [FrqControl == 1]
  state CoordinatedQV [parallel]
    settings: executionOrder=3
    state QVControl_Off
      Mode.VFlag = 0;
    state QVControl_On
      Mode.VFlag = 1;
    (default) -> QVControl_Off
    QVControl_Off -> QVControl_On : [QVControl == 1 && PFControl == 0]
    QVControl_On -> QVControl_Off : [QVControl == 0]
  state PorQ_Priority [parallel]
    settings: executionOrder=4
    state Q_Priority
      Mode.PqFlag = 0;
    state P_Priority
      Mode.PqFlag = 1;
    (default) -> P_Priority
    P_Priority -> Q_Priority : [PQPriority == 0 || QControl == 1]
    Q_Priority -> P_Priority : [PQPriority == 1 && QControl == 0]
  data: QControl input; QVControl input; PFControl input; FrqControl input; PlantControl input; PQPriority input; Mode output Bus: Mode
